simulink model "CLVF"  (R2020a)
settings: Solver=FixedStepAuto  StartTime=0.0  StopTime=tsim  FixedStep=baseRate  RelTol=1e-3  EnableMultiTasking=on
values from neighbouring files (symbols this model uses):
  a = sqrt(sum(aTimesOVec.^2))    [Run_Initializer.m]    (also in a_max_CLVF2D.m = params(4))
  a_max = 0.4/BLACKMass    [Run_Initializer.m]
  a_prime = newParams(2)    [Run_Initializer.m]    (also in a_max_LVF.m = params(2))
  acceptableRadius = 0.05    [Run_Initializer.m]
  b = newParams(3)    [Run_Initializer.m]    (also in a_max_CLVF2D.m = params(3))
  baseRate = 0.05    [Run_Initializer.m]
  BLACKMass = model_param(3)    [Run_Initializer.m]
  d = [0.16;0.542;0]    [Run_Initializer.m]    (also in a_max_LVF.m = [rotStuff(3);rotStuff(4);rotStuff(5)])
  drop_states_BLACK = rC_I0    [Run_Initializer.m]
  drop_states_BLUE = [ xLength/2+0.9; yLength/2+0.5; 0]    [Run_Initializer.m]
  drop_states_RED = rT_I0    [Run_Initializer.m]
  F_thrusters_BLACK = 0.25.*ones(8,1)    [Run_Initializer.m]
  F_thrusters_BLUE = 0.25.*ones(8,1)    [Run_Initializer.m]
  F_thrusters_RED = 0.25.*ones(8,1)    [Run_Initializer.m]
  home_states_BLACK = [ xLength/2+0.4; yLength/2; 0]    [Run_Initializer.m]
  home_states_BLUE = [ xLength/2-0.9; yLength/2+0.5; 0]    [Run_Initializer.m]
  home_states_RED = [ xLength/2-0.4; yLength/2; 0]    [Run_Initializer.m]
  init_states_BLACK = rC_I0    [Run_Initializer.m]
  init_states_BLUE = [ xLength/2+0.9; yLength/2+0.5; 0]    [Run_Initializer.m]
  init_states_RED = rT_I0    [Run_Initializer.m]
  k_v_rel = 2*v_max/a_prime    (= 1)    [Run_Initializer.m]
  ka = newParams(2)    [Run_Initializer.m]    (also in a_max_CLVF2D.m = params(2))
  kc = newParams(1)    [Run_Initializer.m]    (also in a_max_CLVF2D.m = params(1))
  kd = 5.0    (= 5)    [Run_Initializer.m]
  Kd_tb = 0.4    [Run_Initializer.m]
  Kd_tblue = 0.4    [Run_Initializer.m]
  Kd_tr = 0.4    [Run_Initializer.m]
  Kd_xb = 5    [Run_Initializer.m]
  Kd_xblue = 5    [Run_Initializer.m]
  Kd_xr = 5    [Run_Initializer.m]
  Kd_yb = 5    [Run_Initializer.m]
  Kd_yblue = 5    [Run_Initializer.m]
  Kd_yr = 5    [Run_Initializer.m]
  Kp_tb = 0.1    [Run_Initializer.m]
  Kp_tblue = 0.1    [Run_Initializer.m]
  Kp_tr = 0.1    [Run_Initializer.m]
  Kp_xb = 2    [Run_Initializer.m]
  Kp_xblue = 2    [Run_Initializer.m]
  Kp_xr = 2    [Run_Initializer.m]
  Kp_yb = 2    [Run_Initializer.m]
  Kp_yblue = 2    [Run_Initializer.m]
  Kp_yr = 2    [Run_Initializer.m]
  noise_variance_BLACK = 0    [Run_Initializer.m]
  noise_variance_BLUE = 0    [Run_Initializer.m]
  noise_variance_RED = 0    [Run_Initializer.m]
  o_hat_B = aTimesOVec./a    [Run_Initializer.m]
  o_hat_prime = o_prime/sqrt(sum(o_prime.^2))    [Run_Initializer.m]
  Phase0_End = Phase0_Duration    (= 10)    [Run_Initializer.m]
  Phase1_End = Phase0_Duration + Phase1_Duration    (= 15)    [Run_Initializer.m]
  Phase2_End = Phase0_Duration + Phase1_Duration +                                   Phase2_Duration    (= 35)    [Run_Initializer.m]
  Phase3_End = Phase0_Duration + Phase1_Duration +                                   Phase2_Duration + Phase3_Duration    [Run_Initializer.m]
  Phase3_SubPhase1_End = Phase2_End + Phase3_SubPhase1_Duration    (= 40)    [Run_Initializer.m]
  Phase3_SubPhase2_End = Phase2_End + Phase3_SubPhase1_Duration +                                   Phase3_SubPhase2_Duration    (= 45)    [Run_Initializer.m]
  Phase3_SubPhase3_End_BLACK = Phase2_End + Phase3_SubPhase1_Duration +                                   Phase3_SubPhase2_Duration +                                  Phase3_SubPhase3_Duration + Phase3_SubPhase3_and_a_half    (= 51)    [Run_Initializer.m]
  Phase3_SubPhase3_End_RED = Phase2_End + Phase3_SubPhase1_Duration +                                   Phase3_SubPhase2_Duration +                                  Phase3_SubPhase3_Duration    (= 46)    [Run_Initializer.m]
  Phase3_SubPhase4_End = Phase2_End + Phase3_SubPhase1_Duration +                                   Phase3_SubPhase2_Duration +                                  Phase3_SubPhase3_Duration +                                  Phase3_SubPhase4_Duration + Phase3_SubPhase3_and_a_half    [Run_Initializer.m]
  Phase4_End = Phase0_Duration + Phase1_Duration +                                   Phase2_Duration + Phase3_Duration +                                   Phase4_Duration    [Run_Initializer.m]
  Phase5_End = Phase0_Duration + Phase1_Duration +                                   Phase2_Duration + Phase3_Duration +                                   Phase4_Duration + Phase5_Duration    [Run_Initializer.m]
  r_co = r_co_over_a_prime*a_prime    (= 0.16)    [Run_Initializer.m]
  rC_I0 = [0.9*xLength;yLength/2-0.5;pi/2]    [Run_Initializer.m]
  rT_I0 = [yLength/2;yLength/2;possibleStarts(startingRotation)]    [Run_Initializer.m]
  serverRate = 0.1    [Run_Initializer.m]
  sys_BLACK = c2d(sys_BLACK_CONT, baseRate)    [Run_Initializer.m]
  sys_BLACK_ROT = c2d(sys_BLACK_rot_CONT, baseRate)    [Run_Initializer.m]
  sys_RED = c2d(sys_RED_CONT, baseRate)    [Run_Initializer.m]
  sys_RED_ROT = c2d(sys_RED_rot_CONT, baseRate)    [Run_Initializer.m]
  theta_d = 30*d2r    (= 0.523598775598)    [Run_Initializer.m]    (also in a_max_LVF.m = rotStuff(2))
  thruster_dist2CG_BLACK = [83.42;-52.58;55.94;-60.05;54.08;-53.92;77.06;-55.94]    [Run_Initializer.m]
  thruster_dist2CG_BLUE = [83.42;-52.58;55.94;-60.05;54.08;-53.92;77.06;-55.94]    [Run_Initializer.m]
  thruster_dist2CG_RED = [49.92;-78.08;70.46;-63.54;81.08;-50.42;57.44;-75.96]    [Run_Initializer.m]
  w_body = 6.0 * d2r    (= 0.10471975512)    [Run_Initializer.m]
undefined symbols (not defined in the file or in its folder): DiscIntNeverNeededParam, Discrete, Phase3_SubPhase3_End, platformSelection, simMode, Time, WhoAmI
libraries: dspstat3 x18, dspsigops x14, raspberrypiBasiclib x10, embdlinuxlib x8, simulink x8, ctrlSharedLib x4, mspfiltlib x3, dsparch4 x3, dspswit3 x2, MainLibrary x2, sensehatlib x1
(part 6 of 10)

== system CLVF/Gyroscope & Acceleration Algorithms/Change BLUE Behavior/Fix Initial Bias/Correct GyroZ ==
  In1 : Inport
  Calculate Running Mean : Subsystem  TreatAsAtomicUnit=on
  Compare To Zero1 : simulink/Logic and Bit Operations/Compare To Zero  relop===  OutDataTypeStr=boolean
  Data Store Read1 : DataStoreRead  DataStoreName=BLUE_Rz
  Data Store Read3 : DataStoreRead  DataStoreName=BLUE_IMU_R
  Discrete-Time Integrator1 : DiscreteIntegrator  IntegratorMethod=Integration: Backward Euler  ExternalReset=either  InitialConditionSource=external  SampleTime=-1  ICPrevOutput=DiscIntNeverNeededParam  ICPrevScaledInput=DiscIntNeverNeededParam
  If : If  IfExpression=u1 < 5
  Pass Current Gyro : Subsystem  TreatAsAtomicUnit=on
  RED_Px4 : DataStoreWrite  DataStoreName=BLUE_IMU_Psi
  Subsystem : Subsystem
  Subtract : Sum  Inputs=+-
  Out1 : Outport
  wires:
  Subtract/1 -> Out1/1
  Subsystem/1(Time) -> If/1
  If/2 -> Pass Current Gyro/Action
  In1/1 -> Calculate Running Mean/1(In1), Pass Current Gyro/1(In1)
  If/1 -> Calculate Running Mean/Action
  Calculate Running Mean/1(Out1) -> Subtract/2
  Discrete-Time Integrator1/1 -> RED_Px4/1
  Compare To Zero1/1 -> Discrete-Time Integrator1/2
  Pass Current Gyro/1(Out1) -> Compare To Zero1/1, Subtract/1
  Data Store Read3/1 -> Discrete-Time Integrator1/1
  Data Store Read1/1 -> Discrete-Time Integrator1/3

== system CLVF/Gyroscope & Acceleration Algorithms/Change BLUE Behavior/Fix Initial Bias (Accel)/Correct AccelX ==
  In1 : Inport
  Calculate Running Mean : Subsystem  TreatAsAtomicUnit=on
  If : If  IfExpression=u1 < 5
  Pass Current Accel : Subsystem  TreatAsAtomicUnit=on
  Subsystem : Subsystem
  Subtract : Sum  Inputs=+-
  Out1 : Outport
  wires:
  Subtract/1 -> Out1/1
  Subsystem/1(Time) -> If/1
  If/2 -> Pass Current Accel/Action
  In1/1 -> Calculate Running Mean/1(In1), Pass Current Accel/1(In1)
  If/1 -> Calculate Running Mean/Action
  Pass Current Accel/1(Out1) -> Subtract/1
  Calculate Running Mean/1(Out1) -> Subtract/2

== system CLVF/Gyroscope & Acceleration Algorithms/Change BLUE Behavior/Fix Initial Bias (Accel)/Correct AccelY ==
  In1 : Inport
  Calculate Running Mean : Subsystem  TreatAsAtomicUnit=on
  If : If  IfExpression=u1 < 5
  Pass Current Accel : Subsystem  TreatAsAtomicUnit=on
  Subsystem : Subsystem
  Subtract : Sum  Inputs=+-
  Out1 : Outport
  wires:
  Subtract/1 -> Out1/1
  Subsystem/1(Time) -> If/1
  If/2 -> Pass Current Accel/Action
  In1/1 -> Calculate Running Mean/1(In1), Pass Current Accel/1(In1)
  If/1 -> Calculate Running Mean/Action
  Pass Current Accel/1(Out1) -> Subtract/1
  Calculate Running Mean/1(Out1) -> Subtract/2

== system CLVF/Gyroscope & Acceleration Algorithms/Change BLUE Behavior/Fix Initial Bias (Accel)/Correct AccelZ ==
  In1 : Inport
  Calculate Running Mean : Subsystem  TreatAsAtomicUnit=on
  If : If  IfExpression=u1 < 5
  Pass Current Accel : Subsystem  TreatAsAtomicUnit=on
  Subsystem : Subsystem
  Subtract : Sum  Inputs=+-
  Out1 : Outport
  wires:
  Subtract/1 -> Out1/1
  Subsystem/1(Time) -> If/1
  If/2 -> Pass Current Accel/Action
  In1/1 -> Calculate Running Mean/1(In1), Pass Current Accel/1(In1)
  If/1 -> Calculate Running Mean/Action
  Pass Current Accel/1(Out1) -> Subtract/1
  Calculate Running Mean/1(Out1) -> Subtract/2

== system CLVF/Gyroscope & Acceleration Algorithms/Change RED Behavior/Fix Initial Bias/Correct GyroX ==
  In1 : Inport
  Calculate Running Mean : Subsystem  TreatAsAtomicUnit=on
  If : If  IfExpression=u1 < 5
  Pass Current Gyro : Subsystem  TreatAsAtomicUnit=on
  Subsystem : Subsystem
  Subtract : Sum  Inputs=+-
  Out1 : Outport
  wires:
  Subtract/1 -> Out1/1
  Subsystem/1(Time) -> If/1
  If/2 -> Pass Current Gyro/Action
  In1/1 -> Calculate Running Mean/1(In1), Pass Current Gyro/1(In1)
  If/1 -> Calculate Running Mean/Action
  Pass Current Gyro/1(Out1) -> Subtract/1
  Calculate Running Mean/1(Out1) -> Subtract/2

== system CLVF/Gyroscope & Acceleration Algorithms/Change RED Behavior/Fix Initial Bias/Correct GyroY ==
  In1 : Inport
  Calculate Running Mean : Subsystem  TreatAsAtomicUnit=on
  If : If  IfExpression=u1 < 5
  Pass Current Gyro : Subsystem  TreatAsAtomicUnit=on
  Subsystem : Subsystem
  Subtract : Sum  Inputs=+-
  Out1 : Outport
  wires:
  Subtract/1 -> Out1/1
  Subsystem/1(Time) -> If/1
  If/2 -> Pass Current Gyro/Action
  In1/1 -> Calculate Running Mean/1(In1), Pass Current Gyro/1(In1)
  If/1 -> Calculate Running Mean/Action
  Pass Current Gyro/1(Out1) -> Subtract/1
  Calculate Running Mean/1(Out1) -> Subtract/2

== system CLVF/Gyroscope & Acceleration Algorithms/Change RED Behavior/Fix Initial Bias/Correct GyroZ ==
  In1 : Inport
  Calculate Running Mean : Subsystem  TreatAsAtomicUnit=on
  Compare To Zero1 : simulink/Logic and Bit Operations/Compare To Zero  relop===  OutDataTypeStr=boolean
  Data Store Read1 : DataStoreRead  DataStoreName=RED_Rz
  Data Store Read3 : DataStoreRead  DataStoreName=RED_IMU_R
  Discrete-Time Integrator1 : DiscreteIntegrator  IntegratorMethod=Integration: Backward Euler  ExternalReset=either  InitialConditionSource=external  SampleTime=-1  ICPrevOutput=DiscIntNeverNeededParam  ICPrevScaledInput=DiscIntNeverNeededParam
  If : If  IfExpression=u1 < 5
  Pass Current Gyro : Subsystem  TreatAsAtomicUnit=on
  RED_Px4 : DataStoreWrite  DataStoreName=RED_IMU_Psi
  Subsystem : Subsystem
  Subtract : Sum  Inputs=+-
  Out1 : Outport
  wires:
  Subtract/1 -> Out1/1
  Subsystem/1(Time) -> If/1
  If/2 -> Pass Current Gyro/Action
  In1/1 -> Calculate Running Mean/1(In1), Pass Current Gyro/1(In1)
  If/1 -> Calculate Running Mean/Action
  Calculate Running Mean/1(Out1) -> Subtract/2
  Discrete-Time Integrator1/1 -> RED_Px4/1
  Compare To Zero1/1 -> Discrete-Time Integrator1/2
  Pass Current Gyro/1(Out1) -> Compare To Zero1/1, Subtract/1
  Data Store Read3/1 -> Discrete-Time Integrator1/1
  Data Store Read1/1 -> Discrete-Time Integrator1/3

== system CLVF/Gyroscope & Acceleration Algorithms/Change RED Behavior/Fix Initial Bias (Accel)/Correct AccelX ==
  In1 : Inport
  Calculate Running Mean : Subsystem  TreatAsAtomicUnit=on
  If : If  IfExpression=u1 < 5
  Pass Current Accel : Subsystem  TreatAsAtomicUnit=on
  Subsystem : Subsystem
  Subtract : Sum  Inputs=+-
  Out1 : Outport
  wires:
  Subtract/1 -> Out1/1
  Subsystem/1(Time) -> If/1
  If/2 -> Pass Current Accel/Action
  In1/1 -> Calculate Running Mean/1(In1), Pass Current Accel/1(In1)
  If/1 -> Calculate Running Mean/Action
  Pass Current Accel/1(Out1) -> Subtract/1
  Calculate Running Mean/1(Out1) -> Subtract/2

== system CLVF/Gyroscope & Acceleration Algorithms/Change RED Behavior/Fix Initial Bias (Accel)/Correct AccelY ==
  In1 : Inport
  Calculate Running Mean : Subsystem  TreatAsAtomicUnit=on
  If : If  IfExpression=u1 < 5
  Pass Current Accel : Subsystem  TreatAsAtomicUnit=on
  Subsystem : Subsystem
  Subtract : Sum  Inputs=+-
  Out1 : Outport
  wires:
  Subtract/1 -> Out1/1
  Subsystem/1(Time) -> If/1
  If/2 -> Pass Current Accel/Action
  In1/1 -> Calculate Running Mean/1(In1), Pass Current Accel/1(In1)
  If/1 -> Calculate Running Mean/Action
  Pass Current Accel/1(Out1) -> Subtract/1
  Calculate Running Mean/1(Out1) -> Subtract/2

== system CLVF/Gyroscope & Acceleration Algorithms/Change RED Behavior/Fix Initial Bias (Accel)/Correct AccelZ ==
  In1 : Inport
  Calculate Running Mean : Subsystem  TreatAsAtomicUnit=on
  If : If  IfExpression=u1 < 5
  Pass Current Accel : Subsystem  TreatAsAtomicUnit=on
  Subsystem : Subsystem
  Subtract : Sum  Inputs=+-
  Out1 : Outport
  wires:
  Subtract/1 -> Out1/1
  Subsystem/1(Time) -> If/1
  If/2 -> Pass Current Accel/Action
  In1/1 -> Calculate Running Mean/1(In1), Pass Current Accel/1(In1)
  If/1 -> Calculate Running Mean/Action
  Pass Current Accel/1(Out1) -> Subtract/1
  Calculate Running Mean/1(Out1) -> Subtract/2

== system CLVF/Phase #2: Move to Initial Position/Change BLACK Behavior/Custom Discrete PD (Attitude)/x_dot -> x1 ==
  note: dy/dt ~= (y2-y1)/deltaT
  y(t) : Inport
  Delay1 : Delay  DelayLength=1  InitialConditionSource=Input port
      settings: InputPortMap=u0,p4
  Hold this value : Subsystem  TreatAsAtomicUnit=on
  Sum6 : Sum  Inputs=-+|
  divide by delta T : Gain  Gain=1/serverRate
  "if we went through a \"step\"" : If  IfExpression=u1 ~= 0  ShowElse=off
  dy(t)/dt : Outport  VectorParamsAs1DForOutWhenUnconnected=off
  wires:
  divide by delta T/1 -> dy(t)/dt/1
  Delay1/1 -> Sum6/1
  "if we went through a \"step\""/1 -> Hold this value/Action
  Hold this value/1(Out1) -> divide by delta T/1
  Sum6/1 -> "if we went through a \"step\""/1, Hold this value/1(In1)
  y(t)/1 -> Sum6/2, Delay1/2, Delay1/1

== system CLVF/Phase #2: Move to Initial Position/Change BLACK Behavior/Custom Discrete PD (X-Position)/x_dot -> x1 ==
  note: dy/dt ~= (y2-y1)/deltaT
  y(t) : Inport
  Delay1 : Delay  DelayLength=1  InitialConditionSource=Input port
      settings: InputPortMap=u0,p4
  Hold this value : Subsystem  TreatAsAtomicUnit=on
  Sum6 : Sum  Inputs=-+|
  divide by delta T : Gain  Gain=1/serverRate
  "if we went through a \"step\"" : If  IfExpression=u1 ~= 0  ShowElse=off
  dy(t)/dt : Outport  VectorParamsAs1DForOutWhenUnconnected=off
  wires:
  divide by delta T/1 -> dy(t)/dt/1
  Delay1/1 -> Sum6/1
  "if we went through a \"step\""/1 -> Hold this value/Action
  Hold this value/1(Out1) -> divide by delta T/1
  Sum6/1 -> "if we went through a \"step\""/1, Hold this value/1(In1)
  y(t)/1 -> Sum6/2, Delay1/2, Delay1/1

== system CLVF/Phase #2: Move to Initial Position/Change BLACK Behavior/Custom Discrete PD (Y-Position)/x_dot -> x1 ==
  note: dy/dt ~= (y2-y1)/deltaT
  y(t) : Inport
  Delay1 : Delay  DelayLength=1  InitialConditionSource=Input port
      settings: InputPortMap=u0,p4
  Hold this value : Subsystem  TreatAsAtomicUnit=on
  Sum6 : Sum  Inputs=-+|
  divide by delta T : Gain  Gain=1/serverRate
  "if we went through a \"step\"" : If  IfExpression=u1 ~= 0  ShowElse=off
  dy(t)/dt : Outport  VectorParamsAs1DForOutWhenUnconnected=off
  wires:
  divide by delta T/1 -> dy(t)/dt/1
  Delay1/1 -> Sum6/1
  "if we went through a \"step\""/1 -> Hold this value/Action
  Hold this value/1(Out1) -> divide by delta T/1
  Sum6/1 -> "if we went through a \"step\""/1, Hold this value/1(In1)
  y(t)/1 -> Sum6/2, Delay1/2, Delay1/1

== system CLVF/Phase #2: Move to Initial Position/Change BLUE Behavior/Custom Discrete PD (Attitude)/x_dot -> x1 ==
  note: dy/dt ~= (y2-y1)/deltaT
  y(t) : Inport
  Delay1 : Delay  DelayLength=1  InitialConditionSource=Input port
      settings: InputPortMap=u0,p4
  Hold this value : Subsystem  TreatAsAtomicUnit=on
  Sum6 : Sum  Inputs=-+|
  divide by delta T : Gain  Gain=1/serverRate
  "if we went through a \"step\"" : If  IfExpression=u1 ~= 0  ShowElse=off
  dy(t)/dt : Outport  VectorParamsAs1DForOutWhenUnconnected=off
  wires:
  divide by delta T/1 -> dy(t)/dt/1
  Delay1/1 -> Sum6/1
  "if we went through a \"step\""/1 -> Hold this value/Action
  Hold this value/1(Out1) -> divide by delta T/1
  Sum6/1 -> "if we went through a \"step\""/1, Hold this value/1(In1)
  y(t)/1 -> Sum6/2, Delay1/2, Delay1/1

== system CLVF/Phase #2: Move to Initial Position/Change BLUE Behavior/Custom Discrete PD (X-Position)/x_dot -> x1 ==
  note: dy/dt ~= (y2-y1)/deltaT
  y(t) : Inport
  Delay1 : Delay  DelayLength=1  InitialConditionSource=Input port
      settings: InputPortMap=u0,p4
  Hold this value : Subsystem  TreatAsAtomicUnit=on
  Sum6 : Sum  Inputs=-+|
  divide by delta T : Gain  Gain=1/serverRate
  "if we went through a \"step\"" : If  IfExpression=u1 ~= 0  ShowElse=off
  dy(t)/dt : Outport  VectorParamsAs1DForOutWhenUnconnected=off
  wires:
  divide by delta T/1 -> dy(t)/dt/1
  Delay1/1 -> Sum6/1
  "if we went through a \"step\""/1 -> Hold this value/Action
  Hold this value/1(Out1) -> divide by delta T/1
  Sum6/1 -> "if we went through a \"step\""/1, Hold this value/1(In1)
  y(t)/1 -> Sum6/2, Delay1/2, Delay1/1

== system CLVF/Phase #2: Move to Initial Position/Change BLUE Behavior/Custom Discrete PD (Y-Position)/x_dot -> x1 ==
  note: dy/dt ~= (y2-y1)/deltaT
  y(t) : Inport
  Delay1 : Delay  DelayLength=1  InitialConditionSource=Input port
      settings: InputPortMap=u0,p4
  Hold this value : Subsystem  TreatAsAtomicUnit=on
  Sum6 : Sum  Inputs=-+|
  divide by delta T : Gain  Gain=1/serverRate
  "if we went through a \"step\"" : If  IfExpression=u1 ~= 0  ShowElse=off
  dy(t)/dt : Outport  VectorParamsAs1DForOutWhenUnconnected=off
  wires:
  divide by delta T/1 -> dy(t)/dt/1
  Delay1/1 -> Sum6/1
  "if we went through a \"step\""/1 -> Hold this value/Action
  Hold this value/1(Out1) -> divide by delta T/1
  Sum6/1 -> "if we went through a \"step\""/1, Hold this value/1(In1)
  y(t)/1 -> Sum6/2, Delay1/2, Delay1/1

== system CLVF/Phase #2: Move to Initial Position/Change RED Behavior/Custom Discrete PD (Attitude)/x_dot -> x1 ==
  note: dy/dt ~= (y2-y1)/deltaT
  y(t) : Inport
  Delay1 : Delay  DelayLength=1  InitialConditionSource=Input port
      settings: InputPortMap=u0,p4
  Hold this value : Subsystem  TreatAsAtomicUnit=on
  Sum6 : Sum  Inputs=-+|
  divide by delta T : Gain  Gain=1/serverRate
  "if we went through a \"step\"" : If  IfExpression=u1 ~= 0  ShowElse=off
  dy(t)/dt : Outport  VectorParamsAs1DForOutWhenUnconnected=off
  wires:
  divide by delta T/1 -> dy(t)/dt/1
  Delay1/1 -> Sum6/1
  "if we went through a \"step\""/1 -> Hold this value/Action
  Hold this value/1(Out1) -> divide by delta T/1
  Sum6/1 -> "if we went through a \"step\""/1, Hold this value/1(In1)
  y(t)/1 -> Sum6/2, Delay1/2, Delay1/1

== system CLVF/Phase #2: Move to Initial Position/Change RED Behavior/Custom Discrete PD (X-Position)/x_dot -> x1 ==
  note: dy/dt ~= (y2-y1)/deltaT
  y(t) : Inport
  Delay1 : Delay  DelayLength=1  InitialConditionSource=Input port
      settings: InputPortMap=u0,p4
  Hold this value : Subsystem  TreatAsAtomicUnit=on
  Sum6 : Sum  Inputs=-+|
  divide by delta T : Gain  Gain=1/serverRate
  "if we went through a \"step\"" : If  IfExpression=u1 ~= 0  ShowElse=off
  dy(t)/dt : Outport  VectorParamsAs1DForOutWhenUnconnected=off
  wires:
  divide by delta T/1 -> dy(t)/dt/1
  Delay1/1 -> Sum6/1
  "if we went through a \"step\""/1 -> Hold this value/Action
  Hold this value/1(Out1) -> divide by delta T/1
  Sum6/1 -> "if we went through a \"step\""/1, Hold this value/1(In1)
  y(t)/1 -> Sum6/2, Delay1/2, Delay1/1

== system CLVF/Phase #2: Move to Initial Position/Change RED Behavior/Custom Discrete PD (Y-Position)/x_dot -> x1 ==
  note: dy/dt ~= (y2-y1)/deltaT
  y(t) : Inport
  Delay1 : Delay  DelayLength=1  InitialConditionSource=Input port
      settings: InputPortMap=u0,p4
  Hold this value : Subsystem  TreatAsAtomicUnit=on
  Sum6 : Sum  Inputs=-+|
  divide by delta T : Gain  Gain=1/serverRate
  "if we went through a \"step\"" : If  IfExpression=u1 ~= 0  ShowElse=off
  dy(t)/dt : Outport  VectorParamsAs1DForOutWhenUnconnected=off
  wires:
  divide by delta T/1 -> dy(t)/dt/1
  Delay1/1 -> Sum6/1
  "if we went through a \"step\""/1 -> Hold this value/Action
  Hold this value/1(Out1) -> divide by delta T/1
  Sum6/1 -> "if we went through a \"step\""/1, Hold this value/1(In1)
  y(t)/1 -> Sum6/2, Delay1/2, Delay1/1

== system CLVF/Phase #3: Experiment/Change BLACK Behavior/Sub-Phase #1/Custom Discrete PD (Attitude) ==
  ez : Inport
  Sum3 : Sum
  kd_tb : Gain  Gain=Kd_tb
  kp_tb : Gain  Gain=Kp_tb
  "x_dot -> x1" : Subsystem
  Tz : Outport  VectorParamsAs1DForOutWhenUnconnected=off
  wires:
  kd_tb/1 -> Sum3/1
  Sum3/1 -> Tz/1
  kp_tb/1 -> Sum3/2
  "x_dot -> x1"/1(dy(t)/dt) -> kd_tb/1
  ez/1 -> "x_dot -> x1"/1(y(t)), kp_tb/1

== system CLVF/Phase #3: Experiment/Change BLACK Behavior/Sub-Phase #1/Custom Discrete PD (X-Position) ==
  ex : Inport
  Sum3 : Sum
  kd_xb : Gain  Gain=Kd_xb
  kp_xb : Gain  Gain=Kp_xb
  "x_dot -> x1" : Subsystem
  Fx : Outport  VectorParamsAs1DForOutWhenUnconnected=off
  wires:
  kd_xb/1 -> Sum3/1
  ex/1 -> "x_dot -> x1"/1(y(t)), kp_xb/1
  kp_xb/1 -> Sum3/2
  "x_dot -> x1"/1(dy(t)/dt) -> kd_xb/1
  Sum3/1 -> Fx/1

== system CLVF/Phase #3: Experiment/Change BLACK Behavior/Sub-Phase #1/Custom Discrete PD (Y-Position) ==
  ey : Inport
  Sum3 : Sum
  kd_yb : Gain  Gain=Kd_yb
  kp_yb : Gain  Gain=Kp_yb
  "x_dot -> x1" : Subsystem
  Fy : Outport  VectorParamsAs1DForOutWhenUnconnected=off
  wires:
  kd_yb/1 -> Sum3/1
  Sum3/1 -> Fy/1
  kp_yb/1 -> Sum3/2
  "x_dot -> x1"/1(dy(t)/dt) -> kd_yb/1
  ey/1 -> "x_dot -> x1"/1(y(t)), kp_yb/1

== system CLVF/Phase #3: Experiment/Change BLACK Behavior/Sub-Phase #1/Hough Control ==
  Ref : Inport
  Act : Inport  Port=2
  MATLAB Function2 : MATLAB Function  TreatAsAtomicUnit=on
  MATLAB Function3 : MATLAB Function  TreatAsAtomicUnit=on
  MATLAB Function4 : MATLAB Function  TreatAsAtomicUnit=on
  Subtract2 : Sum  Inputs=+-
  Err : Outport  VectorParamsAs1DForOutWhenUnconnected=off
  wires:
  MATLAB Function4/1(e_out) -> Err/1
  MATLAB Function2/1(Oy) -> MATLAB Function4/1(Oy)
  Subtract2/1 -> MATLAB Function4/2(e_in)
  MATLAB Function2/2(Ox) -> Subtract2/1
  Act/1 -> MATLAB Function3/1(z)
  Ref/1 -> MATLAB Function2/1(z)
  MATLAB Function3/1(Ox) -> Subtract2/2

== system CLVF/Phase #3: Experiment/Change BLACK Behavior/Sub-Phase #4/BLACK_RzD ==
  Desired Rate (BLACK) : Constant  Value=0.104719755/2  SampleTime=-1
  Product : Product
  Subsystem : Subsystem
  Wrap1 : Subsystem
  Out1 : Outport  VectorParamsAs1DForOutWhenUnconnected=off
  wires:
  Wrap1/1(wrapped) -> Out1/1
  Desired Rate (BLACK)/1 -> Product/1
  Subsystem/1(Time) -> Product/2
  Product/1 -> Wrap1/1(unwrapped)

== system CLVF/Phase #3: Experiment/Change BLACK Behavior/Sub-Phase #4/Custom Discrete PD (Attitude) ==
  ez : Inport
  Sum3 : Sum
  kd_tb : Gain  Gain=Kd_tb
  kp_tb : Gain  Gain=Kp_tb
  "x_dot -> x1" : Subsystem
  Tz : Outport  VectorParamsAs1DForOutWhenUnconnected=off
  wires:
  kd_tb/1 -> Sum3/1
  Sum3/1 -> Tz/1
  kp_tb/1 -> Sum3/2
  "x_dot -> x1"/1(dy(t)/dt) -> kd_tb/1
  ez/1 -> "x_dot -> x1"/1(y(t)), kp_tb/1

== system CLVF/Phase #3: Experiment/Change BLACK Behavior/Sub-Phase #4/Hough Control ==
  Ref : Inport
  Act : Inport  Port=2
  MATLAB Function2 : MATLAB Function  TreatAsAtomicUnit=on
  MATLAB Function3 : MATLAB Function  TreatAsAtomicUnit=on
  MATLAB Function4 : MATLAB Function  TreatAsAtomicUnit=on
  Subtract2 : Sum  Inputs=+-
  Err : Outport  VectorParamsAs1DForOutWhenUnconnected=off
  wires:
  MATLAB Function4/1(e_out) -> Err/1
  MATLAB Function2/1(Oy) -> MATLAB Function4/1(Oy)
  Subtract2/1 -> MATLAB Function4/2(e_in)
  MATLAB Function2/2(Ox) -> Subtract2/1
  Act/1 -> MATLAB Function3/1(z)
  Ref/1 -> MATLAB Function2/1(z)
  MATLAB Function3/1(Ox) -> Subtract2/2

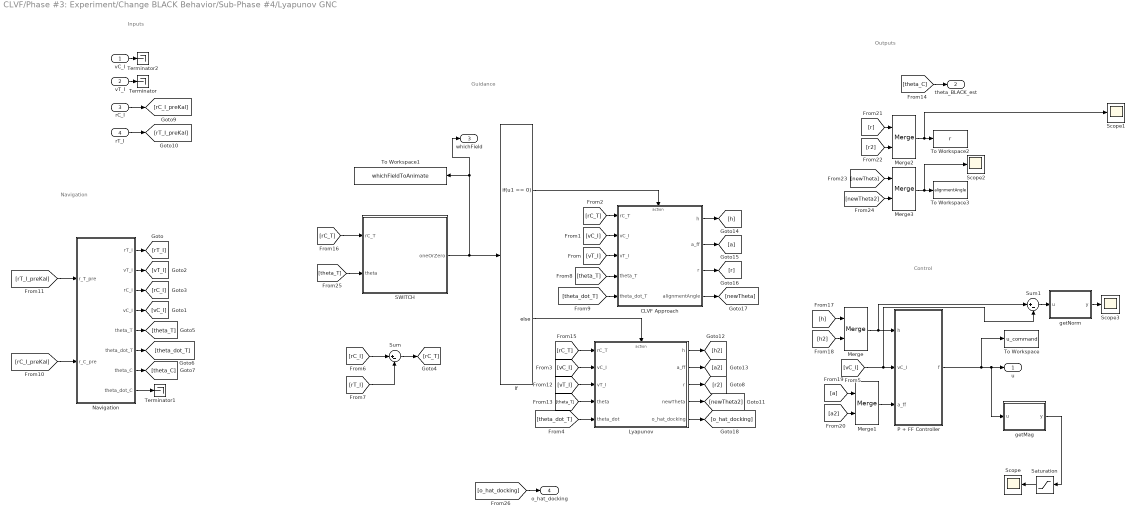
== system CLVF/Phase #3: Experiment/Change BLACK Behavior/Sub-Phase #4/Lyapunov GNC ==
  note: Inputs
  note: Outputs
  note: Navigation
  note: Guidance
  note: Control
  vC_I : Inport
  vT_I : Inport  Port=2
  rC_I : Inport  Port=3
  rT_I : Inport  Port=4
  CLVF Approach : Subsystem
  If : If  IfExpression=u1 == 0
  Lyapunov : Subsystem  TreatAsAtomicUnit=on
  Merge{,1..3} (4 alike) : Merge
  Navigation : Subsystem
  P + FF Controller : MATLAB Function  TreatAsAtomicUnit=on
  SWITCH : Subsystem
  Saturation : Saturate  UpperLimit=a_max*BLACKMass  LowerLimit=0
  Scope{,1..3} (4 alike) : Scope
  Sum : Sum  Inputs=|+-
  Sum1 : Sum  Inputs=|+-
  Terminator : Terminator
  Terminator1 : Terminator
  Terminator2 : Terminator
  To Workspace : ToWorkspace  VariableName=u_command  SampleTime=-1
  To Workspace1 : ToWorkspace  VariableName=whichFieldToAnimate  SampleTime=-1
  To Workspace2 : ToWorkspace  VariableName=r  SampleTime=-1
  To Workspace3 : ToWorkspace  VariableName=alignmentAngle  SampleTime=-1
  getMag : MATLAB Function  TreatAsAtomicUnit=on
  getNorm : MATLAB Function  TreatAsAtomicUnit=on
  u : Outport  VectorParamsAs1DForOutWhenUnconnected=off
  theta_BLACK_est : Outport  Port=2  VectorParamsAs1DForOutWhenUnconnected=off
  whichField : Outport  Port=3  VectorParamsAs1DForOutWhenUnconnected=off
  o_hat_docking : Outport  Port=4  VectorParamsAs1DForOutWhenUnconnected=off
  wires:
  P + FF Controller/1(f) -> To Workspace/1, getMag/1(u), u/1
  [vT_I] -> CLVF Approach/3(vT_I)
  [vC_I] -> CLVF Approach/2(vC_I)
  [rC_T] -> CLVF Approach/1(rC_T)
  If/1 -> CLVF Approach/Action
  If/2 -> Lyapunov/Action
  SWITCH/1(oneOrZero) -> To Workspace1/1, whichField/1, If/1
  [rC_I] -> Sum/1
  [rT_I] -> Sum/2
  Sum/1 -> [rC_T]
  vC_I/1 -> Terminator2/1
  vT_I/1 -> Terminator/1
  [theta_T] -> CLVF Approach/4(theta_T)
  [theta_dot_T] -> CLVF Approach/5(theta_dot_T)
  getMag/1(y) -> Saturation/1
  Saturation/1 -> Scope/1
  rT_I/1 -> [rT_I_preKal]
  rC_I/1 -> [rC_I_preKal]
  [theta_C] -> theta_BLACK_est/1
  [rC_I_preKal] -> Navigation/2(r_C_pre)
  [rT_I_preKal] -> Navigation/1(r_T_pre)
  Navigation/1(rT_I) -> [rT_I]
  Navigation/4(vC_I) -> [vC_I]
  Navigation/2(vT_I) -> [vT_I]
  Navigation/3(rC_I) -> [rC_I]
  Navigation/5(theta_T) -> [theta_T]
  Navigation/6(theta_dot_T) -> [theta_dot_T]
  Navigation/7(theta_C) -> [theta_C]
  Navigation/8(theta_dot_C) -> Terminator1/1
  Lyapunov/2(a_ff) -> [a2]
  Lyapunov/4(newTheta) -> [newTheta2]
  [rC_T] -> Lyapunov/1(rC_T)
  [theta_dot_T] -> Lyapunov/5(theta_dot)
  [vC_I] -> Lyapunov/2(vC_I)
  [vT_I] -> Lyapunov/3(vT_I)
  [theta_T] -> Lyapunov/4(theta)
  Lyapunov/1(h) -> [h2]
  Lyapunov/3(r) -> [r2]
  [vC_I] -> Sum1/2, P + FF Controller/2(vC_I)
  [theta_T] -> SWITCH/2(theta)
  [rC_T] -> SWITCH/1(rC_T)
  CLVF Approach/1(h) -> [h]
  CLVF Approach/2(a_ff) -> [a]
  CLVF Approach/3(r) -> [r]
  CLVF Approach/4(alignmentAngle) -> [newTheta]
  Merge/1 -> Sum1/1, P + FF Controller/1(h)
  [h] -> Merge/1
  [h2] -> Merge/2
  [a] -> Merge1/1
  [a2] -> Merge1/2
  Merge1/1 -> P + FF Controller/3(a_ff)
  [r] -> Merge2/1
  [r2] -> Merge2/2
  Merge2/1 -> Scope1/1, To Workspace2/1
  [newTheta2] -> Merge3/2
  [newTheta] -> Merge3/1
  Lyapunov/5(o_hat_docking) -> [o_hat_docking]
  [o_hat_docking] -> o_hat_docking/1
  Merge3/1 -> Scope2/1, To Workspace3/1
  Sum1/1 -> getNorm/1(u)
  getNorm/1(y) -> Scope3/1

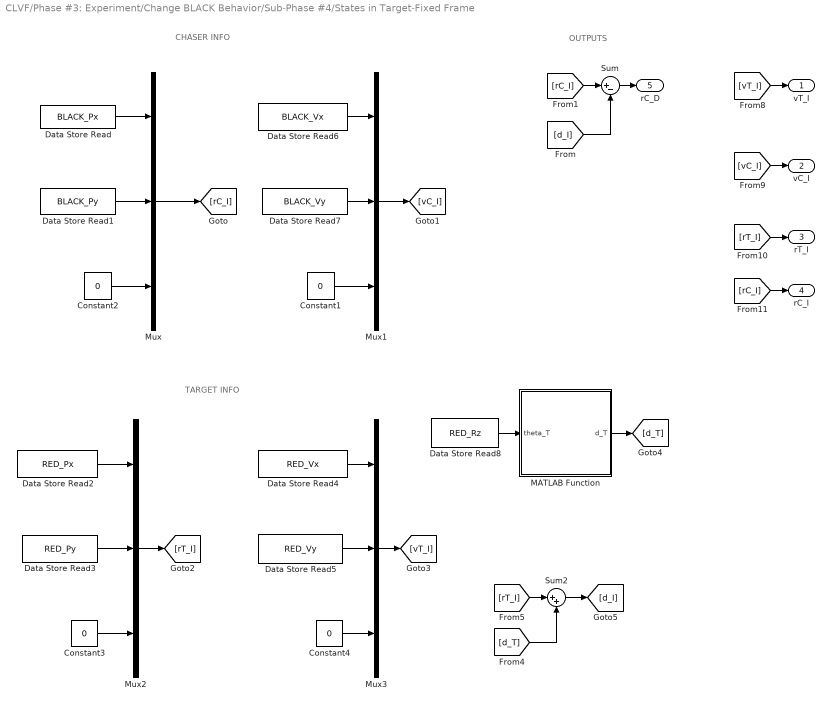
== system CLVF/Phase #3: Experiment/Change BLACK Behavior/Sub-Phase #4/States in Target-Fixed Frame ==
  note: OUTPUTS
  note: CHASER INFO
  note: TARGET INFO
  Constant{1..4} (4 alike) : Constant  Value=0
  Data Store Read : DataStoreRead  DataStoreName=BLACK_Px
  Data Store Read1 : DataStoreRead  DataStoreName=BLACK_Py
  Data Store Read2 : DataStoreRead  DataStoreName=RED_Px
  Data Store Read3 : DataStoreRead  DataStoreName=RED_Py
  Data Store Read4 : DataStoreRead  DataStoreName=RED_Vx
  Data Store Read5 : DataStoreRead  DataStoreName=RED_Vy
  Data Store Read6 : DataStoreRead  DataStoreName=BLACK_Vx
  Data Store Read7 : DataStoreRead  DataStoreName=BLACK_Vy
  Data Store Read8 : DataStoreRead  DataStoreName=RED_Rz
  MATLAB Function : MATLAB Function  TreatAsAtomicUnit=on
  Mux{,1..3} (4 alike) : Mux  Inputs=3
  Sum : Sum  Inputs=|+-
  Sum2 : Sum  Inputs=|++
  vT_I : Outport  VectorParamsAs1DForOutWhenUnconnected=off
  vC_I : Outport  Port=2  VectorParamsAs1DForOutWhenUnconnected=off
  rT_I : Outport  Port=3  VectorParamsAs1DForOutWhenUnconnected=off
  rC_I : Outport  Port=4  VectorParamsAs1DForOutWhenUnconnected=off
  rC_D : Outport  Port=5  VectorParamsAs1DForOutWhenUnconnected=off
  wires:
  Data Store Read/1 -> Mux/1
  Data Store Read1/1 -> Mux/2
  Constant2/1 -> Mux/3
  Data Store Read7/1 -> Mux1/2
  Data Store Read6/1 -> Mux1/1
  Constant1/1 -> Mux1/3
  Mux/1 -> [rC_I]
  Mux1/1 -> [vC_I]
  Data Store Read2/1 -> Mux2/1
  Data Store Read3/1 -> Mux2/2
  Constant3/1 -> Mux2/3
  Mux2/1 -> [rT_I]
  Mux3/1 -> [vT_I]
  Data Store Read4/1 -> Mux3/1
  Data Store Read5/1 -> Mux3/2
  Constant4/1 -> Mux3/3
  Data Store Read8/1 -> MATLAB Function/1(theta_T)
  MATLAB Function/1(d_T) -> [d_T]
  [d_T] -> Sum2/2
  [rT_I] -> Sum2/1
  Sum2/1 -> [d_I]
  [vT_I] -> vT_I/1
  [vC_I] -> vC_I/1
  [rT_I] -> rT_I/1
  [rC_I] -> rC_I/1
  Sum/1 -> rC_D/1
  [rC_I] -> Sum/1
  [d_I] -> Sum/2

== system CLVF/Phase #3: Experiment/Change BLUE Behavior/Sub-Phase #1/Custom Discrete PD (Attitude) ==
  ez : Inport
  Sum3 : Sum
  kd_tb : Gain  Gain=Kd_tblue
  kp_tb : Gain  Gain=Kp_tblue
  "x_dot -> x1" : Subsystem
  Tz : Outport  VectorParamsAs1DForOutWhenUnconnected=off
  wires:
  kd_tb/1 -> Sum3/1
  Sum3/1 -> Tz/1
  kp_tb/1 -> Sum3/2
  "x_dot -> x1"/1(dy(t)/dt) -> kd_tb/1
  ez/1 -> "x_dot -> x1"/1(y(t)), kp_tb/1

== system CLVF/Phase #3: Experiment/Change BLUE Behavior/Sub-Phase #1/Custom Discrete PD (X-Position) ==
  ex : Inport
  Sum3 : Sum
  kd_xb : Gain  Gain=Kd_xblue
  kp_xb : Gain  Gain=Kp_xblue
  "x_dot -> x1" : Subsystem
  Fx : Outport  VectorParamsAs1DForOutWhenUnconnected=off
  wires:
  kd_xb/1 -> Sum3/1
  ex/1 -> "x_dot -> x1"/1(y(t)), kp_xb/1
  kp_xb/1 -> Sum3/2
  "x_dot -> x1"/1(dy(t)/dt) -> kd_xb/1
  Sum3/1 -> Fx/1

== system CLVF/Phase #3: Experiment/Change BLUE Behavior/Sub-Phase #1/Custom Discrete PD (Y-Position) ==
  ey : Inport
  Sum3 : Sum
  kd_yb : Gain  Gain=Kd_yblue
  kp_yb : Gain  Gain=Kp_yblue
  "x_dot -> x1" : Subsystem
  Fy : Outport  VectorParamsAs1DForOutWhenUnconnected=off
  wires:
  kd_yb/1 -> Sum3/1
  Sum3/1 -> Fy/1
  kp_yb/1 -> Sum3/2
  "x_dot -> x1"/1(dy(t)/dt) -> kd_yb/1
  ey/1 -> "x_dot -> x1"/1(y(t)), kp_yb/1

== system CLVF/Phase #3: Experiment/Change BLUE Behavior/Sub-Phase #1/Hough Control ==
  Ref : Inport
  Act : Inport  Port=2
  MATLAB Function2 : MATLAB Function  TreatAsAtomicUnit=on
  MATLAB Function3 : MATLAB Function  TreatAsAtomicUnit=on
  MATLAB Function4 : MATLAB Function  TreatAsAtomicUnit=on
  Subtract2 : Sum  Inputs=+-
  Err : Outport  VectorParamsAs1DForOutWhenUnconnected=off
  wires:
  MATLAB Function4/1(e_out) -> Err/1
  MATLAB Function2/1(Oy) -> MATLAB Function4/1(Oy)
  Subtract2/1 -> MATLAB Function4/2(e_in)
  MATLAB Function2/2(Ox) -> Subtract2/1
  Act/1 -> MATLAB Function3/1(z)
  Ref/1 -> MATLAB Function2/1(z)
  MATLAB Function3/1(Ox) -> Subtract2/2

== system CLVF/Phase #3: Experiment/Change BLUE Behavior/Sub-Phase #4/Custom Discrete PD (Attitude) ==
  ez : Inport
  Sum3 : Sum
  kd_tb : Gain  Gain=Kd_tblue
  kp_tb : Gain  Gain=Kp_tblue
  "x_dot -> x1" : Subsystem
  Tz : Outport  VectorParamsAs1DForOutWhenUnconnected=off
  wires:
  kd_tb/1 -> Sum3/1
  Sum3/1 -> Tz/1
  kp_tb/1 -> Sum3/2
  "x_dot -> x1"/1(dy(t)/dt) -> kd_tb/1
  ez/1 -> "x_dot -> x1"/1(y(t)), kp_tb/1

== system CLVF/Phase #3: Experiment/Change BLUE Behavior/Sub-Phase #4/Custom Discrete PD (X-Position) ==
  ex : Inport
  Sum3 : Sum
  kd_xb : Gain  Gain=Kd_xblue
  kp_xb : Gain  Gain=Kp_xblue
  "x_dot -> x1" : Subsystem
  Fx : Outport  VectorParamsAs1DForOutWhenUnconnected=off
  wires:
  kd_xb/1 -> Sum3/1
  ex/1 -> "x_dot -> x1"/1(y(t)), kp_xb/1
  kp_xb/1 -> Sum3/2
  "x_dot -> x1"/1(dy(t)/dt) -> kd_xb/1
  Sum3/1 -> Fx/1

== system CLVF/Phase #3: Experiment/Change BLUE Behavior/Sub-Phase #4/Custom Discrete PD (Y-Position) ==
  ey : Inport
  Sum3 : Sum
  kd_yb : Gain  Gain=Kd_yblue
  kp_yb : Gain  Gain=Kp_yblue
  "x_dot -> x1" : Subsystem
  Fy : Outport  VectorParamsAs1DForOutWhenUnconnected=off
  wires:
  kd_yb/1 -> Sum3/1
  Sum3/1 -> Fy/1
  kp_yb/1 -> Sum3/2
  "x_dot -> x1"/1(dy(t)/dt) -> kd_yb/1
  ey/1 -> "x_dot -> x1"/1(y(t)), kp_yb/1

== system CLVF/Phase #3: Experiment/Change BLUE Behavior/Sub-Phase #4/Hough Control ==
  Ref : Inport
  Act : Inport  Port=2
  MATLAB Function2 : MATLAB Function  TreatAsAtomicUnit=on
  MATLAB Function3 : MATLAB Function  TreatAsAtomicUnit=on
  MATLAB Function4 : MATLAB Function  TreatAsAtomicUnit=on
  Subtract2 : Sum  Inputs=+-
  Err : Outport  VectorParamsAs1DForOutWhenUnconnected=off
  wires:
  MATLAB Function4/1(e_out) -> Err/1
  MATLAB Function2/1(Oy) -> MATLAB Function4/1(Oy)
  Subtract2/1 -> MATLAB Function4/2(e_in)
  MATLAB Function2/2(Ox) -> Subtract2/1
  Act/1 -> MATLAB Function3/1(z)
  Ref/1 -> MATLAB Function2/1(z)
  MATLAB Function3/1(Ox) -> Subtract2/2

== system CLVF/Phase #3: Experiment/Change RED Behavior/Sub-Phase #1/Custom Discrete PD (Attitude) ==
  ez : Inport
  Sum3 : Sum
  kd_tr : Gain  Gain=Kd_tr
  kp_tr : Gain  Gain=Kp_tr
  "x_dot -> x1" : Subsystem
  Tz : Outport  VectorParamsAs1DForOutWhenUnconnected=off
  wires:
  kd_tr/1 -> Sum3/1
  Sum3/1 -> Tz/1
  kp_tr/1 -> Sum3/2
  "x_dot -> x1"/1(dy(t)/dt) -> kd_tr/1
  ez/1 -> "x_dot -> x1"/1(y(t)), kp_tr/1

== system CLVF/Phase #3: Experiment/Change RED Behavior/Sub-Phase #1/Custom Discrete PD (X-Position) ==
  ex : Inport
  Sum3 : Sum
  kd_xr : Gain  Gain=Kd_xr
  kp_xr : Gain  Gain=Kp_xr
  "x_dot -> x1" : Subsystem
  Fx : Outport  VectorParamsAs1DForOutWhenUnconnected=off
  wires:
  kd_xr/1 -> Sum3/1
  ex/1 -> "x_dot -> x1"/1(y(t)), kp_xr/1
  kp_xr/1 -> Sum3/2
  "x_dot -> x1"/1(dy(t)/dt) -> kd_xr/1
  Sum3/1 -> Fx/1

== system CLVF/Phase #3: Experiment/Change RED Behavior/Sub-Phase #1/Custom Discrete PD (Y-Position) ==
  ey : Inport
  Sum3 : Sum
  kd_yr : Gain  Gain=Kd_yr
  kp_yr : Gain  Gain=Kp_yr
  "x_dot -> x1" : Subsystem
  Fy : Outport  VectorParamsAs1DForOutWhenUnconnected=off
  wires:
  kd_yr/1 -> Sum3/1
  Sum3/1 -> Fy/1
  kp_yr/1 -> Sum3/2
  "x_dot -> x1"/1(dy(t)/dt) -> kd_yr/1
  ey/1 -> "x_dot -> x1"/1(y(t)), kp_yr/1

== system CLVF/Phase #3: Experiment/Change RED Behavior/Sub-Phase #1/Hough Control ==
  Ref : Inport
  Act : Inport  Port=2
  MATLAB Function2 : MATLAB Function  TreatAsAtomicUnit=on
  MATLAB Function3 : MATLAB Function  TreatAsAtomicUnit=on
  MATLAB Function4 : MATLAB Function  TreatAsAtomicUnit=on
  Subtract2 : Sum  Inputs=+-
  Err : Outport  VectorParamsAs1DForOutWhenUnconnected=off
  wires:
  MATLAB Function4/1(e_out) -> Err/1
  MATLAB Function2/1(Oy) -> MATLAB Function4/1(Oy)
  Subtract2/1 -> MATLAB Function4/2(e_in)
  MATLAB Function2/2(Ox) -> Subtract2/1
  Act/1 -> MATLAB Function3/1(z)
  Ref/1 -> MATLAB Function2/1(z)
  MATLAB Function3/1(Ox) -> Subtract2/2

== system CLVF/Phase #3: Experiment/Change RED Behavior/Sub-Phase #4/Custom Discrete PD (Attitude) ==
  ez : Inport
  Sum3 : Sum
  kd_tr : Gain  Gain=Kd_tr
  kp_tr : Gain  Gain=Kp_tr
  "x_dot -> x1" : Subsystem
  Tz : Outport  VectorParamsAs1DForOutWhenUnconnected=off
  wires:
  kd_tr/1 -> Sum3/1
  Sum3/1 -> Tz/1
  kp_tr/1 -> Sum3/2
  "x_dot -> x1"/1(dy(t)/dt) -> kd_tr/1
  ez/1 -> "x_dot -> x1"/1(y(t)), kp_tr/1

== system CLVF/Phase #3: Experiment/Change RED Behavior/Sub-Phase #4/Custom Discrete PD (X-Position) ==
  ex : Inport
  Sum3 : Sum
  kd_xr : Gain  Gain=Kd_xr
  kp_xr : Gain  Gain=Kp_xr
  "x_dot -> x1" : Subsystem
  Fx : Outport  VectorParamsAs1DForOutWhenUnconnected=off
  wires:
  kd_xr/1 -> Sum3/1
  ex/1 -> "x_dot -> x1"/1(y(t)), kp_xr/1
  kp_xr/1 -> Sum3/2
  "x_dot -> x1"/1(dy(t)/dt) -> kd_xr/1
  Sum3/1 -> Fx/1

== system CLVF/Phase #3: Experiment/Change RED Behavior/Sub-Phase #4/Custom Discrete PD (Y-Position) ==
  ey : Inport
  Sum3 : Sum
  kd_yr : Gain  Gain=Kd_yr
  kp_yr : Gain  Gain=Kp_yr
  "x_dot -> x1" : Subsystem
  Fy : Outport  VectorParamsAs1DForOutWhenUnconnected=off
  wires:
  kd_yr/1 -> Sum3/1
  Sum3/1 -> Fy/1
  kp_yr/1 -> Sum3/2
  "x_dot -> x1"/1(dy(t)/dt) -> kd_yr/1
  ey/1 -> "x_dot -> x1"/1(y(t)), kp_yr/1

== system CLVF/Phase #3: Experiment/Change RED Behavior/Sub-Phase #4/Hough Control ==
  Ref : Inport
  Act : Inport  Port=2
  MATLAB Function2 : MATLAB Function  TreatAsAtomicUnit=on
  MATLAB Function3 : MATLAB Function  TreatAsAtomicUnit=on
  MATLAB Function4 : MATLAB Function  TreatAsAtomicUnit=on
  Subtract2 : Sum  Inputs=+-
  Err : Outport  VectorParamsAs1DForOutWhenUnconnected=off
  wires:
  MATLAB Function4/1(e_out) -> Err/1
  MATLAB Function2/1(Oy) -> MATLAB Function4/1(Oy)
  Subtract2/1 -> MATLAB Function4/2(e_in)
  MATLAB Function2/2(Ox) -> Subtract2/1
  Act/1 -> MATLAB Function3/1(z)
  Ref/1 -> MATLAB Function2/1(z)
  MATLAB Function3/1(Ox) -> Subtract2/2

== system CLVF/Phase #3: Experiment/Change RED Behavior/Sub-Phase #4/Subsystem ==
  Constant1 : Constant  Value=Phase3_SubPhase3_End_RED  SampleTime=-1
  Subtract : Sum  Inputs=+-
  Universal_Time : DataStoreRead  DataStoreName=Univ_Time
  Time : Outport  VectorParamsAs1DForOutWhenUnconnected=off
  wires:
  Universal_Time/1 -> Subtract/1
  Subtract/1 -> Time/1
  Constant1/1 -> Subtract/2

== system CLVF/Phase #4: Return Home/Change BLACK Behavior/Custom Discrete PD (Attitude)/x_dot -> x1 ==
  note: dy/dt ~= (y2-y1)/deltaT
  y(t) : Inport
  Delay1 : Delay  DelayLength=1  InitialConditionSource=Input port
      settings: InputPortMap=u0,p4
  Hold this value : Subsystem  TreatAsAtomicUnit=on
  Sum6 : Sum  Inputs=-+|
  divide by delta T : Gain  Gain=1/serverRate
  "if we went through a \"step\"" : If  IfExpression=u1 ~= 0  ShowElse=off
  dy(t)/dt : Outport  VectorParamsAs1DForOutWhenUnconnected=off
  wires:
  divide by delta T/1 -> dy(t)/dt/1
  Delay1/1 -> Sum6/1
  "if we went through a \"step\""/1 -> Hold this value/Action
  Hold this value/1(Out1) -> divide by delta T/1
  Sum6/1 -> "if we went through a \"step\""/1, Hold this value/1(In1)
  y(t)/1 -> Sum6/2, Delay1/2, Delay1/1

== system CLVF/Phase #4: Return Home/Change BLACK Behavior/Custom Discrete PD (X-Position)/x_dot -> x1 ==
  note: dy/dt ~= (y2-y1)/deltaT
  y(t) : Inport
  Delay1 : Delay  DelayLength=1  InitialConditionSource=Input port
      settings: InputPortMap=u0,p4
  Hold this value : Subsystem  TreatAsAtomicUnit=on
  Sum6 : Sum  Inputs=-+|
  divide by delta T : Gain  Gain=1/serverRate
  "if we went through a \"step\"" : If  IfExpression=u1 ~= 0  ShowElse=off
  dy(t)/dt : Outport  VectorParamsAs1DForOutWhenUnconnected=off
  wires:
  divide by delta T/1 -> dy(t)/dt/1
  Delay1/1 -> Sum6/1
  "if we went through a \"step\""/1 -> Hold this value/Action
  Hold this value/1(Out1) -> divide by delta T/1
  Sum6/1 -> "if we went through a \"step\""/1, Hold this value/1(In1)
  y(t)/1 -> Sum6/2, Delay1/2, Delay1/1

== system CLVF/Phase #4: Return Home/Change BLACK Behavior/Custom Discrete PD (Y-Position)/x_dot -> x1 ==
  note: dy/dt ~= (y2-y1)/deltaT
  y(t) : Inport
  Delay1 : Delay  DelayLength=1  InitialConditionSource=Input port
      settings: InputPortMap=u0,p4
  Hold this value : Subsystem  TreatAsAtomicUnit=on
  Sum6 : Sum  Inputs=-+|
  divide by delta T : Gain  Gain=1/serverRate
  "if we went through a \"step\"" : If  IfExpression=u1 ~= 0  ShowElse=off
  dy(t)/dt : Outport  VectorParamsAs1DForOutWhenUnconnected=off
  wires:
  divide by delta T/1 -> dy(t)/dt/1
  Delay1/1 -> Sum6/1
  "if we went through a \"step\""/1 -> Hold this value/Action
  Hold this value/1(Out1) -> divide by delta T/1
  Sum6/1 -> "if we went through a \"step\""/1, Hold this value/1(In1)
  y(t)/1 -> Sum6/2, Delay1/2, Delay1/1

== system CLVF/Phase #4: Return Home/Change BLUE Behavior/Custom Discrete PD (Attitude)/x_dot -> x1 ==
  note: dy/dt ~= (y2-y1)/deltaT
  y(t) : Inport
  Delay1 : Delay  DelayLength=1  InitialConditionSource=Input port
      settings: InputPortMap=u0,p4
  Hold this value : Subsystem  TreatAsAtomicUnit=on
  Sum6 : Sum  Inputs=-+|
  divide by delta T : Gain  Gain=1/serverRate
  "if we went through a \"step\"" : If  IfExpression=u1 ~= 0  ShowElse=off
  dy(t)/dt : Outport  VectorParamsAs1DForOutWhenUnconnected=off
  wires:
  divide by delta T/1 -> dy(t)/dt/1
  Delay1/1 -> Sum6/1
  "if we went through a \"step\""/1 -> Hold this value/Action
  Hold this value/1(Out1) -> divide by delta T/1
  Sum6/1 -> "if we went through a \"step\""/1, Hold this value/1(In1)
  y(t)/1 -> Sum6/2, Delay1/2, Delay1/1

== system CLVF/Phase #4: Return Home/Change BLUE Behavior/Custom Discrete PD (X-Position)/x_dot -> x1 ==
  note: dy/dt ~= (y2-y1)/deltaT
  y(t) : Inport
  Delay1 : Delay  DelayLength=1  InitialConditionSource=Input port
      settings: InputPortMap=u0,p4
  Hold this value : Subsystem  TreatAsAtomicUnit=on
  Sum6 : Sum  Inputs=-+|
  divide by delta T : Gain  Gain=1/serverRate
  "if we went through a \"step\"" : If  IfExpression=u1 ~= 0  ShowElse=off
  dy(t)/dt : Outport  VectorParamsAs1DForOutWhenUnconnected=off
  wires:
  divide by delta T/1 -> dy(t)/dt/1
  Delay1/1 -> Sum6/1
  "if we went through a \"step\""/1 -> Hold this value/Action
  Hold this value/1(Out1) -> divide by delta T/1
  Sum6/1 -> "if we went through a \"step\""/1, Hold this value/1(In1)
  y(t)/1 -> Sum6/2, Delay1/2, Delay1/1

== system CLVF/Phase #4: Return Home/Change BLUE Behavior/Custom Discrete PD (Y-Position)/x_dot -> x1 ==
  note: dy/dt ~= (y2-y1)/deltaT
  y(t) : Inport
  Delay1 : Delay  DelayLength=1  InitialConditionSource=Input port
      settings: InputPortMap=u0,p4
  Hold this value : Subsystem  TreatAsAtomicUnit=on
  Sum6 : Sum  Inputs=-+|
  divide by delta T : Gain  Gain=1/serverRate
  "if we went through a \"step\"" : If  IfExpression=u1 ~= 0  ShowElse=off
  dy(t)/dt : Outport  VectorParamsAs1DForOutWhenUnconnected=off
  wires:
  divide by delta T/1 -> dy(t)/dt/1
  Delay1/1 -> Sum6/1
  "if we went through a \"step\""/1 -> Hold this value/Action
  Hold this value/1(Out1) -> divide by delta T/1
  Sum6/1 -> "if we went through a \"step\""/1, Hold this value/1(In1)
  y(t)/1 -> Sum6/2, Delay1/2, Delay1/1

== system CLVF/Phase #4: Return Home/Change RED Behavior/Custom Discrete PD (Attitude)/x_dot -> x1 ==
  note: dy/dt ~= (y2-y1)/deltaT
  y(t) : Inport
  Delay1 : Delay  DelayLength=1  InitialConditionSource=Input port
      settings: InputPortMap=u0,p4
  Hold this value : Subsystem  TreatAsAtomicUnit=on
  Sum6 : Sum  Inputs=-+|
  divide by delta T : Gain  Gain=1/serverRate
  "if we went through a \"step\"" : If  IfExpression=u1 ~= 0  ShowElse=off
  dy(t)/dt : Outport  VectorParamsAs1DForOutWhenUnconnected=off
  wires:
  divide by delta T/1 -> dy(t)/dt/1
  Delay1/1 -> Sum6/1
  "if we went through a \"step\""/1 -> Hold this value/Action
  Hold this value/1(Out1) -> divide by delta T/1
  Sum6/1 -> "if we went through a \"step\""/1, Hold this value/1(In1)
  y(t)/1 -> Sum6/2, Delay1/2, Delay1/1

== system CLVF/Phase #4: Return Home/Change RED Behavior/Custom Discrete PD (X-Position)/x_dot -> x1 ==
  note: dy/dt ~= (y2-y1)/deltaT
  y(t) : Inport
  Delay1 : Delay  DelayLength=1  InitialConditionSource=Input port
      settings: InputPortMap=u0,p4
  Hold this value : Subsystem  TreatAsAtomicUnit=on
  Sum6 : Sum  Inputs=-+|
  divide by delta T : Gain  Gain=1/serverRate
  "if we went through a \"step\"" : If  IfExpression=u1 ~= 0  ShowElse=off
  dy(t)/dt : Outport  VectorParamsAs1DForOutWhenUnconnected=off
  wires:
  divide by delta T/1 -> dy(t)/dt/1
  Delay1/1 -> Sum6/1
  "if we went through a \"step\""/1 -> Hold this value/Action
  Hold this value/1(Out1) -> divide by delta T/1
  Sum6/1 -> "if we went through a \"step\""/1, Hold this value/1(In1)
  y(t)/1 -> Sum6/2, Delay1/2, Delay1/1

== system CLVF/Phase #4: Return Home/Change RED Behavior/Custom Discrete PD (Y-Position)/x_dot -> x1 ==
  note: dy/dt ~= (y2-y1)/deltaT
  y(t) : Inport
  Delay1 : Delay  DelayLength=1  InitialConditionSource=Input port
      settings: InputPortMap=u0,p4
  Hold this value : Subsystem  TreatAsAtomicUnit=on
  Sum6 : Sum  Inputs=-+|
  divide by delta T : Gain  Gain=1/serverRate
  "if we went through a \"step\"" : If  IfExpression=u1 ~= 0  ShowElse=off
  dy(t)/dt : Outport  VectorParamsAs1DForOutWhenUnconnected=off
  wires:
  divide by delta T/1 -> dy(t)/dt/1
  Delay1/1 -> Sum6/1
  "if we went through a \"step\""/1 -> Hold this value/Action
  Hold this value/1(Out1) -> divide by delta T/1
  Sum6/1 -> "if we went through a \"step\""/1, Hold this value/1(In1)
  y(t)/1 -> Sum6/2, Delay1/2, Delay1/1

== system CLVF/Phase #5: Hold Home/Change BLACK Behavior/Custom Discrete PD (Attitude)/x_dot -> x1 ==
  note: dy/dt ~= (y2-y1)/deltaT
  y(t) : Inport
  Delay1 : Delay  DelayLength=1  InitialConditionSource=Input port
      settings: InputPortMap=u0,p4
  Hold this value : Subsystem  TreatAsAtomicUnit=on
  Sum6 : Sum  Inputs=-+|
  divide by delta T : Gain  Gain=1/serverRate
  "if we went through a \"step\"" : If  IfExpression=u1 ~= 0  ShowElse=off
  dy(t)/dt : Outport  VectorParamsAs1DForOutWhenUnconnected=off
  wires:
  divide by delta T/1 -> dy(t)/dt/1
  Delay1/1 -> Sum6/1
  "if we went through a \"step\""/1 -> Hold this value/Action
  Hold this value/1(Out1) -> divide by delta T/1
  Sum6/1 -> "if we went through a \"step\""/1, Hold this value/1(In1)
  y(t)/1 -> Sum6/2, Delay1/2, Delay1/1

== system CLVF/Phase #5: Hold Home/Change BLACK Behavior/Custom Discrete PD (X-Position)/x_dot -> x1 ==
  note: dy/dt ~= (y2-y1)/deltaT
  y(t) : Inport
  Delay1 : Delay  DelayLength=1  InitialConditionSource=Input port
      settings: InputPortMap=u0,p4
  Hold this value : Subsystem  TreatAsAtomicUnit=on
  Sum6 : Sum  Inputs=-+|
  divide by delta T : Gain  Gain=1/serverRate
  "if we went through a \"step\"" : If  IfExpression=u1 ~= 0  ShowElse=off
  dy(t)/dt : Outport  VectorParamsAs1DForOutWhenUnconnected=off
  wires:
  divide by delta T/1 -> dy(t)/dt/1
  Delay1/1 -> Sum6/1
  "if we went through a \"step\""/1 -> Hold this value/Action
  Hold this value/1(Out1) -> divide by delta T/1
  Sum6/1 -> "if we went through a \"step\""/1, Hold this value/1(In1)
  y(t)/1 -> Sum6/2, Delay1/2, Delay1/1

== system CLVF/Phase #5: Hold Home/Change BLACK Behavior/Custom Discrete PD (Y-Position)/x_dot -> x1 ==
  note: dy/dt ~= (y2-y1)/deltaT
  y(t) : Inport
  Delay1 : Delay  DelayLength=1  InitialConditionSource=Input port
      settings: InputPortMap=u0,p4
  Hold this value : Subsystem  TreatAsAtomicUnit=on
  Sum6 : Sum  Inputs=-+|
  divide by delta T : Gain  Gain=1/serverRate
  "if we went through a \"step\"" : If  IfExpression=u1 ~= 0  ShowElse=off
  dy(t)/dt : Outport  VectorParamsAs1DForOutWhenUnconnected=off
  wires:
  divide by delta T/1 -> dy(t)/dt/1
  Delay1/1 -> Sum6/1
  "if we went through a \"step\""/1 -> Hold this value/Action
  Hold this value/1(Out1) -> divide by delta T/1
  Sum6/1 -> "if we went through a \"step\""/1, Hold this value/1(In1)
  y(t)/1 -> Sum6/2, Delay1/2, Delay1/1

== system CLVF/Phase #5: Hold Home/Change BLUE Behavior/Custom Discrete PD (Attitude)/x_dot -> x1 ==
  note: dy/dt ~= (y2-y1)/deltaT
  y(t) : Inport
  Delay1 : Delay  DelayLength=1  InitialConditionSource=Input port
      settings: InputPortMap=u0,p4
  Hold this value : Subsystem  TreatAsAtomicUnit=on
  Sum6 : Sum  Inputs=-+|
  divide by delta T : Gain  Gain=1/serverRate
  "if we went through a \"step\"" : If  IfExpression=u1 ~= 0  ShowElse=off
  dy(t)/dt : Outport  VectorParamsAs1DForOutWhenUnconnected=off
  wires:
  divide by delta T/1 -> dy(t)/dt/1
  Delay1/1 -> Sum6/1
  "if we went through a \"step\""/1 -> Hold this value/Action
  Hold this value/1(Out1) -> divide by delta T/1
  Sum6/1 -> "if we went through a \"step\""/1, Hold this value/1(In1)
  y(t)/1 -> Sum6/2, Delay1/2, Delay1/1

== system CLVF/Phase #5: Hold Home/Change BLUE Behavior/Custom Discrete PD (X-Position)/x_dot -> x1 ==
  note: dy/dt ~= (y2-y1)/deltaT
  y(t) : Inport
  Delay1 : Delay  DelayLength=1  InitialConditionSource=Input port
      settings: InputPortMap=u0,p4
  Hold this value : Subsystem  TreatAsAtomicUnit=on
  Sum6 : Sum  Inputs=-+|
  divide by delta T : Gain  Gain=1/serverRate
  "if we went through a \"step\"" : If  IfExpression=u1 ~= 0  ShowElse=off
  dy(t)/dt : Outport  VectorParamsAs1DForOutWhenUnconnected=off
  wires:
  divide by delta T/1 -> dy(t)/dt/1
  Delay1/1 -> Sum6/1
  "if we went through a \"step\""/1 -> Hold this value/Action
  Hold this value/1(Out1) -> divide by delta T/1
  Sum6/1 -> "if we went through a \"step\""/1, Hold this value/1(In1)
  y(t)/1 -> Sum6/2, Delay1/2, Delay1/1
